simulink model "spherical_wrist"  (R2023b)
settings: Solver=VariableStepAuto  StartTime=0.0  StopTime=20  FixedStep=0.001  RelTol=1e-3
InitFcn:
  | WRIST_60_50_DataFile
model workspace (MAT data in the model file):
  Damp = Simulink.Parameter
  Damp.Value = 0.0001
  Damp.DataType = 'auto'
  Damp.Complexity = 'real'
  Damp.Dimensions = [1 1]
  Dm = Simulink.Parameter
  Dm.Value = 7.4e-05
  Dm.DataType = 'auto'
  Dm.DocUnits = 'mN*m/rpm'
  Dm.Complexity = 'real'
  Dm.Dimensions = [1 1]
  Jm = Simulink.Parameter
  Jm.Value = 3.3
  Jm.DataType = 'auto'
  Jm.DocUnits = 'g*cm^2'
  Jm.Complexity = 'real'
  Jm.Dimensions = [1 1]
  Km = Simulink.Parameter
  Km.Value = 32.2
  Km.DataType = 'auto'
  Km.DocUnits = 'mN*m/A'
  Km.Complexity = 'real'
  Km.Dimensions = [1 1]
  Tc = Simulink.Parameter
  Tc.Value = 0.001
  Tc.DataType = 'auto'
  Tc.DocUnits = 's'
  Tc.Complexity = 'real'
  Tc.Dimensions = [1 1]
values from neighbouring files (symbols this model uses):
  PQ = [P(1,:)*Q(1,:)' P(2,:)*Q(2,:)' P(3,:)*Q(3,:)']    [WRIST_60_50_DataFile.m]
  Pz = -tand(30)*[1; 1; 1]    [WRIST_60_50_DataFile.m]
  Q = [cosd(plat_off) sind(plat_off) [0; 0; 0]]    [WRIST_60_50_DataFile.m]
undefined symbols (not defined in the file or in its folder): smiData, X, Y, Z
libraries: sm_lib x44, nesl_utility x20, fl_lib x15, sdl_lib x9, sharedtransform x2, slpidlib x1
(part 1 of 3)
settings Model: Creator=ascalzo  LastModifiedBy=upattacini
settings SolverCC: AlgebraicLoopSolver=TrustRegion
settings OptimizationCC: DefaultParameterBehavior=Inlined  UseDivisionForNetSlopeComputation=on  GainParamInheritBuiltInType=on  UseFloatMulNetSlope=on  InlineInvariantSignals=on  ReuseModelBlockBuffer=off  PassReuseOutputArgsAs=Individual arguments  ZeroExternalMemoryAtStartup=off  ZeroInternalMemoryAtStartup=off  NoFixptDivByZeroProtection=on  EfficientFloat2IntCast=on  LifeSpan=1  OptimizeBlockOrder=speed  DifferentSizesBufferReuse=on  EfficientTunableParamExpr=on
settings DebuggingCC: ParameterTunabilityLossMsg=error  UnconnectedInputMsg=warning  UnconnectedOutputMsg=warning  UnconnectedLineMsg=warning
settings HardwareCC: ProdBitPerPointer=32  ProdBitPerSizeT=32  ProdBitPerPtrDiffT=32  ProdLargestAtomicInteger=Long  ProdLargestAtomicFloat=Double  ProdWordSize=32  ProdLongLongMode=on  ProdHWDeviceType=ARM Compatible->ARM Cortex-M
settings ModelReferenceCC: EnableRefExpFcnMdlSchedulingChecks=on
settings SFSimCC: MATLABDynamicMemAlloc=off  SimTargetLang=C++
settings RTWCC: Description=Embedded Coder  SystemTargetFile=ert.tlc  GenCodeOnly=on  PackageGeneratedCodeAndArtifacts=on  PackageName=WristDecoupler.zip  TemplateMakefile=ert_default_tmf  GenerateReport=on  Toolchain=Microsoft Visual C++ 2019 v16.0 | nmake (64-bit Windows)  LaunchReport=on  TargetLang=C++  DLArmComputeVersion=19.05
settings CodeAppCC: ForceParamTrailComments=on  IgnoreCustomStorageClasses=off  OperatorAnnotations=on  SimulinkDataObjDesc=on  SFDataObjDesc=on  CustomSymbolStrGlobalVar=rt$N$M  CustomSymbolStrType=$N$M  CustomSymbolStrFcn=$N$M$F  CustomSymbolStrMacro=$N$M  InsertBlockDesc=on  MATLABSourceComments=on
settings ERTTargetCC: TargetLangStandard=C++03 (ISO)  GenerateSampleERTMain=on  IncludeMdlTerminateFcn=off  CombineSignalStateStructs=on  CodeInterfacePackaging=C++ class  SupportComplex=off  SupportNonInlinedSFcns=on  InlinedParameterPlacement=NonHierarchical  RootIOFormat=Structure reference  ERTCustomFileTemplate=example_file_process.tlc  ERTFilePackagingFormat=CompactWithDataFile

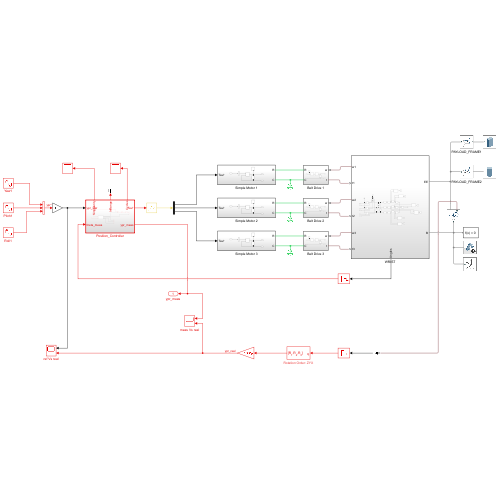
[thumbnail: Simulink's stored preview of the top-level diagram]
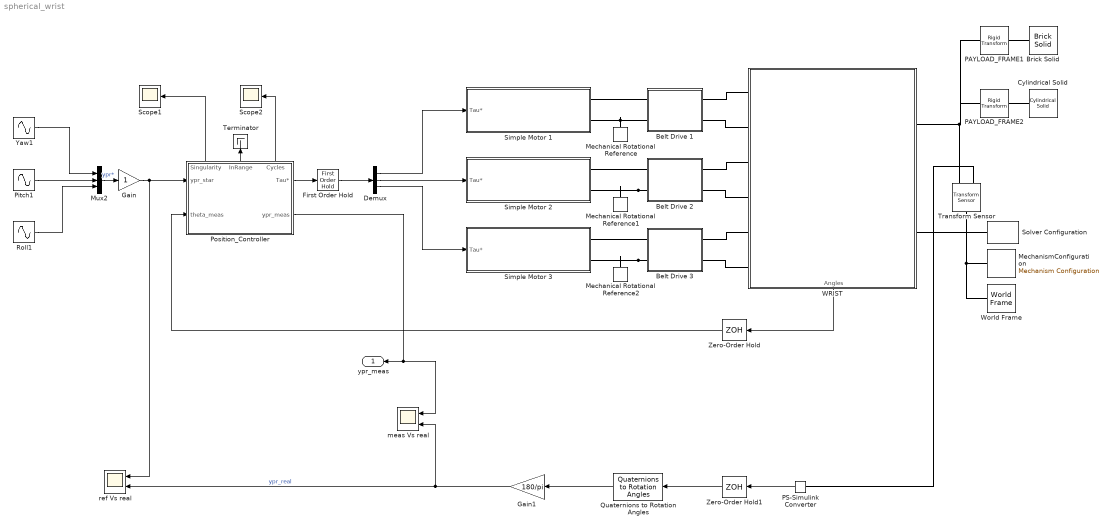
== system spherical_wrist ==
  Belt Drive 1 : Subsystem
  Belt Drive 2 : Subsystem
  Belt Drive 3 : Subsystem
  Brick Solid : sm_lib/Body Elements/Brick Solid  GraphicAmbientColor=[0.15 0.15 0.15 1.0]  BasedOnType=Density  BrickDimensions=[50 50 50]  BrickDimensionsUnits=mm  CenterOfMass=[0 0 0]  CenterOfMassUnits=m  GraphicDiffuseColor=[0.5 0.5 0.5]  Density=12000  DensityUnits=kg/m^3  DoExposeReferenceFrame=on  GraphicEmissiveColor=[0.0 0.0 0.0 1.0]  ExportEntireGeometry=off  SerializedFrames=<Frames/>  MarkerShape=Sphere  MarkerSize=10  GraphicType=FromGeometry  InertiaType=CalculateFromGeometry  Mass=1.5  MassUnits=kg  MomentsOfInertia=[1 1 1]  MomentsOfInertiaUnits=kg*m^2  GraphicOpacity=1  ProductsOfInertia=[0 0 0]  ProductsOfInertiaUnits=kg*m^2  GraphicShininess=75  GraphicSpecularColor=[0.5 0.5 0.5 1.0]  GraphicVisPropType=SimpleVisualProperties
  Cylindrical Solid : sm_lib/Body Elements/Cylindrical Solid  GraphicAmbientColor=[0.15 0.15 0.15 1.0]  BasedOnType=Density  CenterOfMass=[0 0 0]  CenterOfMassUnits=m  GraphicDiffuseColor=[0.5 0.5 0.5]  CylinderLength=56  CylinderLengthUnits=mm  CylinderRadius=4  CylinderRadiusUnits=mm  Density=1000  DensityUnits=kg/m^3  DoExposeReferenceFrame=on  GraphicEmissiveColor=[0.0 0.0 0.0 1.0]  ExportEntireGeometry=off  SerializedFrames=<Frames/>  MarkerShape=Sphere  MarkerSize=10  GraphicType=FromGeometry  InertiaType=PointMass  Mass=500  MassUnits=g  MomentsOfInertia=[1 1 1]  MomentsOfInertiaUnits=kg*m^2  GraphicOpacity=1  ProductsOfInertia=[0 0 0]  ProductsOfInertiaUnits=kg*m^2  GraphicShininess=75  GraphicSpecularColor=[0.5 0.5 0.5 1.0]  GraphicVisPropType=SimpleVisualProperties
  Demux : Demux  Outputs=3
  First Order Hold : FirstOrderHold  ErrorTolerance=inf
  Gain : Gain
  Gain1 : Gain  Gain=180/pi
  Mechanical Rotational Reference : fl_lib/Mechanical/Rotational Elements/Mechanical Rotational Reference
  Mechanical Rotational Reference1 : fl_lib/Mechanical/Rotational Elements/Mechanical Rotational Reference
  Mechanical Rotational Reference2 : fl_lib/Mechanical/Rotational Elements/Mechanical Rotational Reference
  MechanismConfiguration : sm_lib/Utilities/Mechanism Configuration  UniformGravity=Constant  GravityVector=[0 0 9.80665]  GravityVectorUnits=m/s^2  LinearizationDelta=0.001  JointModeTransitionNonlinearIterations=2
  Mux2 : Mux  Inputs=3
  PAYLOAD_FRAME1 : sm_lib/Frames and Transforms/Rigid Transform  TranslationMethod=Cartesian  TranslationStandardOffset=0  TranslationStandardOffsetUnits=mm  TranslationStandardAxis=+Z  TranslationCartesianOffset=[0 0 70]  TranslationCartesianOffsetUnits=mm  TranslationROffset=0  TranslationROffsetUnits=m  TranslationZOffset=0  TranslationZOffsetUnits=m  TranslationThetaOffset=0  TranslationThetaOffsetUnits=deg  RotationMethod=None  RotationAngleUnits=rad  RotationStandardAxis=+Z  RotationAngle=smiData.RigidTransform(2).angle  RotationArbitraryAxis=smiData.RigidTransform(2).axis  FollAlignAxisA=+X  BaseAlignAxisA=+Y  FollAlignAxisB=+Y  BaseAlignAxisB=+Z  RotationSequenceAxes=FollowerAxes  RotationSequence=XYX  RotationSequenceAngles=[0 0 0]  RotationSequenceAnglesUnits=deg  RotationMatrix=[1 0 0; 0 1 0; 0 0 1]  Quaternion=[1 0 0 0]
  PAYLOAD_FRAME2 : sm_lib/Frames and Transforms/Rigid Transform  TranslationMethod=Cartesian  TranslationStandardOffset=0  TranslationStandardOffsetUnits=mm  TranslationStandardAxis=+Z  TranslationCartesianOffset=[0 0 30]  TranslationCartesianOffsetUnits=mm  TranslationROffset=0  TranslationROffsetUnits=m  TranslationZOffset=0  TranslationZOffsetUnits=m  TranslationThetaOffset=0  TranslationThetaOffsetUnits=deg  RotationMethod=None  RotationAngleUnits=rad  RotationStandardAxis=+Z  RotationAngle=smiData.RigidTransform(2).angle  RotationArbitraryAxis=smiData.RigidTransform(2).axis  FollAlignAxisA=+X  BaseAlignAxisA=+Y  FollAlignAxisB=+Y  BaseAlignAxisB=+Z  RotationSequenceAxes=FollowerAxes  RotationSequence=XYX  RotationSequenceAngles=[0 0 0]  RotationSequenceAnglesUnits=deg  RotationMatrix=[1 0 0; 0 1 0; 0 0 1]  Quaternion=[1 0 0 0]
  PS-Simulink Converter : nesl_utility/PS-Simulink Converter  PhysicalDomain=network_engine_domain  SubClassName=ps_output  LeftPortType=input  RightPortType=output  PseudoPeriodic=off  Frequencies=[]  VectorFormat=1-D array  Unit=inherit  AffineConversion=off
  Pitch1 : Sin  Amplitude=55  Bias=-5  Frequency=60/55  Phase=asin(5/55)  SampleTime=Tc
  Position_Controller : Subsystem  TreatAsAtomicUnit=on  SystemSampleTime=0.001
      settings: MinAlgLoopOccurrences=on  PortSchema="{\"entries\":[{\"content\":{\"sides\":[{\"content\":{\"connectorIds\":[\"In1\",\"In2\"]},\"type\":\"ConnectorPlacement.EquallySpacedRectSide\",\"uuid\":\"83213a6a-d539-4d4b-893d-998d212c9f51\"},{\"content\":{\"connectorIds\":[\"Out1\",\"Out2\"],\"side\":\"RIGHT\"},\"type\":\"ConnectorPlacement.EquallySpacedRectSide\",\"uuid\":\"07d19463-f1b8-4ef2-82ae-a356a5259b0c\"},{\"content\":{\"connectorIds\":[\"Out3\",\"Out4\",\"Out5\"],\"side\":\"TOP\"},\"type\":\"ConnectorPlacement.EquallySpacedRectSide\",\"uuid\":\"262960f5-5579-40eb-9028-5284e67b897c\"}]},\"type\":\"ConnectorPlacement.EquallySpacedConnector\",\"uuid\":\"3a54d725-4b36-4299-8af9-8f83752d9c8a\"}],\"packageUris\":[\"http://schema.mathworks.com/mf0/Connector/19700101\"],\"version\":\"1.0\"}"
  Quaternions to Rotation Angles : sharedtransform/Quaternions to Rotation Angles  rotationOrder=ZYX  aMode=aMode
  Roll1 : Sin  Amplitude=30  Frequency=60/30  SampleTime=Tc
  Scope1 : Scope
  Scope2 : Scope
  Simple Motor 1 : Subsystem
  Simple Motor 2 : Subsystem
  Simple Motor 3 : Subsystem
  Solver Configuration : nesl_utility/Solver Configuration  PhysicalDomain=network_engine_domain  SubClassName=solver  LeftPortType=input  RightPortType=generic  Tones=[]  Harmonics=[]  SimulateNoise=off  Profile=off  UseLocalSampling=off  EnableSwitchedLinearOptims=on  FrequencyDomain=off  UseCCode=off  RelTol=0.001  AbsTol=1e-06  MinStep=1e-09  ToWorkspace=off  RevertToSquareIcSolve=off  NumHomotopyIterations=100  PhasorMode=off  PhasorModeNumHarmonics=1  ConsistencySolver=NEWTON_FTOL  IndexReductionMethod=DerivativeReplacement  DoDC=off  ResidualTolerance=1e-09  ConsistencyTolSource=GLOBAL  ConsistencyAbsTol=0.001  ConsistencyRelTol=0.001  ConsistencyTolFactor=0.001  UseLocalSolver=off  LocalSolverChoice=NE_TRAPEZOIDAL_ADVANCER  ResolveIndetEquations=on  FunctionEvalNumThread=1  LocalSolverSampleTime=0.0001  DoFixedCost=off  MaxNonlinIter=3  MaxModeIter=2  ComputeImpulses=off  ImpulseIterations=2  LinearAlgebra=auto  LinearAlgebraNumThread=0  EquationFormulation=NE_TIME_EF  DelaysMemoryBudget=1024  AutomaticFiltering=on  FilteringTimeConstant=0.001  PartitionStorageMethod=AS_NEEDED  PartitionMemoryBudget=1024  PartitionMethod=ROBUST  MultibodyUseLocalSolver=off  MultibodyLocalSolverChoice=ODE1  MultibodyLocalSolverSampleTime=0.001
  Terminator : Terminator
  Transform Sensor : sm_lib/Frames and Transforms/Transform Sensor  MeasurementFrame=World  RotationSequence=XYX  SenseAngle=off  SenseAxis=off  SenseQ=on  SenseR=off  SenseRotationSequence=off  SenseOmegaX=off  SenseOmegaY=off  SenseOmegaZ=off  SenseOmega=off  SenseQDot=off  SenseRDot=off  SenseRotationSequenceDot=off  SenseAlphaX=off  SenseAlphaY=off  SenseAlphaZ=off  SenseAlpha=off  SenseQDDot=off  SenseRDDot=off  SenseX=off  SenseY=off  SenseZ=off  SenseXYZ=off  SenseRad=off  SenseAzim=off  SenseDist=off  SenseInc=off  SenseXDot=off  SenseYDot=off  SenseZDot=off  SenseXYZDot=off  SenseRadDot=off  SenseAzimDot=off  SenseDistDot=off  SenseIncDot=off  SenseXDDot=off  SenseYDDot=off  SenseZDDot=off  SenseXYZDDot=off  SenseRadDDot=off  SenseAzimDDot=off  SenseDistDDot=off  SenseIncDDot=off
  WRIST : Subsystem
      settings: PortSchema="{\"entries\":[{\"content\":{\"sides\":[{\"content\":{\"connectorIds\":[\"LConn1\",\"LConn2\",\"LConn3\",\"LConn4\",\"LConn5\",\"LConn6\"]},\"type\":\"ConnectorPlacement.EquallySpacedRectSide\",\"uuid\":\"837cba77-e4d8-410a-871c-09f9d5b58985\"},{\"content\":{\"connectorIds\":[\"RConn1\",\"RConn2\"],\"side\":\"RIGHT\"},\"type\":\"ConnectorPlacement.EquallySpacedRectSide\",\"uuid\":\"e99e27fa-5cde-4df4-999c-5c540dbd874f\"},{\"content\":{\"connectorIds\":[],\"side\":\"TOP\"},\"type\":\"ConnectorPlacement.EquallySpacedRectSide\",\"uuid\":\"93dbe70b-6d44-4b10-9b14-70f8e934205d\"},{\"content\":{\"connectorIds\":[\"Out1\"],\"side\":\"BOTTOM\"},\"type\":\"ConnectorPlacement.EquallySpacedRectSide\",\"uuid\":\"bafba6b5-af66-4d82-b4b8-19931a0ab184\"}]},\"type\":\"ConnectorPlacement.EquallySpacedConnector\",\"uuid\":\"c57b24f6-44a7-49b3-8fbc-a4c709c10c31\"}],\"packageUris\":[\"http://schema.mathworks.com/mf0/Connector/19700101\"],\"version\":\"1.0\"}"
  World Frame : sm_lib/Frames and Transforms/World Frame
  Yaw1 : Sin  Amplitude=90  Frequency=60/90  SampleTime=Tc
  Zero-Order Hold : ZeroOrderHold  SampleTime=Tc
  Zero-Order Hold1 : ZeroOrderHold  SampleTime=Tc
  meas Vs real : Scope  NumInputPorts=2
  ref Vs real : Scope  NumInputPorts=2
  ypr_meas : Outport
  wires:
  WRIST/1(Angles) -> Zero-Order Hold/1
  Gain1/1 -> ref Vs real/2, meas Vs real/2  "ypr_real"
  PS-Simulink Converter/1 -> Zero-Order Hold1/1
  Quaternions to Rotation Angles/1 -> Gain1/1
  Yaw1/1 -> Mux2/1
  Mux2/1 -> Gain/1  "ypr*"
  Roll1/1 -> Mux2/3
  Pitch1/1 -> Mux2/2
  Demux/1 -> Simple Motor 1/1(Tau*)
  Demux/2 -> Simple Motor 2/1(Tau*)
  Demux/3 -> Simple Motor 3/1(Tau*)
  First Order Hold/1 -> Demux/1
  Position_Controller/2(ypr_meas) -> meas Vs real/1, ypr_meas/1
  Position_Controller/1(Tau*) -> First Order Hold/1
  Position_Controller/5(Cycles) -> Scope2/1
  Gain/1 -> ref Vs real/1, Position_Controller/1(ypr_star)
  Position_Controller/3(Singularity) -> Scope1/1
  Position_Controller/4(InRange) -> Terminator/1
  Zero-Order Hold/1 -> Position_Controller/2(theta_meas)
  Zero-Order Hold1/1 -> Quaternions to Rotation Angles/1
  connections:
  World Frame/RConn1 -- Solver Configuration/RConn1 -- Transform Sensor/LConn1 -- WRIST/RConn2 -- MechanismConfiguration/RConn1
  PAYLOAD_FRAME1/LConn1 -- PAYLOAD_FRAME2/LConn1 -- Transform Sensor/RConn1 -- WRIST/RConn1
  Transform Sensor/RConn2 -- PS-Simulink Converter/LConn1
  Cylindrical Solid/RConn1 -- PAYLOAD_FRAME2/RConn1
  Brick Solid/RConn1 -- PAYLOAD_FRAME1/RConn1
  WRIST/LConn1 -- Belt Drive 1/RConn1
  Mechanical Rotational Reference/LConn1 -- Simple Motor 1/RConn2 -- Belt Drive 1/LConn2
  Belt Drive 1/LConn1 -- Simple Motor 1/RConn1
  Belt Drive 2/LConn2 -- Simple Motor 2/RConn2 -- Mechanical Rotational Reference1/LConn1
  Belt Drive 2/LConn1 -- Simple Motor 2/RConn1
  WRIST/LConn3 -- Belt Drive 2/RConn1
  Belt Drive 3/LConn2 -- Simple Motor 3/RConn2 -- Mechanical Rotational Reference2/LConn1
  Belt Drive 3/LConn1 -- Simple Motor 3/RConn1
  WRIST/LConn5 -- Belt Drive 3/RConn1
  Belt Drive 1/RConn2 -- WRIST/LConn2
  Belt Drive 2/RConn2 -- WRIST/LConn4
  Belt Drive 3/RConn2 -- WRIST/LConn6

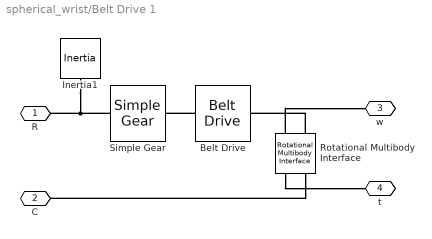
== system spherical_wrist/Belt Drive 1 ==
  Belt Drive : sdl_lib/Couplings & Drives/Belt Drive  drive_type=sdl.enum.wrap_configuration.open  belt_type=sdl.enum.belt_type.ideal  sheave_ang=30 deg  num_belts=1  model_f_c=sdl.enum.model_centrifugal.off  linear_density=0.6 kg/m  model_compliance=sdl.enum.compliance.off  stiffness=1e4 N/m  damping=1e3 N/(m/s)  tension=100 N  breakable=sdl.enum.max_tension.off  F_max=1e5 N  r_pulley_A=14 mm  b_pulley_A=0.1 N*m/(rad/s)  model_inertia_A=sdl.enum.model_inertia.on  pulley_inertia_A=10 g*mm^2  initial_velocity_A=0 rad/s  r_pulley_B=28 mm  b_pulley_B=0.1 N*m/(rad/s)  model_inertia_B=sdl.enum.model_inertia.on  pulley_inertia_B=10 g*mm^2  initial_velocity_B=0 rad/s  friction_model=sdl.enum.PulleyModel.Continuous  initial_state_locked_A=sdl.enum.initial_lock.unlocked  initial_state_locked_B=sdl.enum.initial_lock.unlocked  mu=0.5  mu_static=0.5  mu_kinetic=0.42  wrap_parameterization=sdl.enum.wrap_parameterization.centers  d_centers=0.5 m  phi_wrap_A=145 deg  phi_wrap_B=215 deg  v_thr=0.001 m/s  f_thr=1 N
      settings: InternalSimscapePortConfiguration="{\"Bottom\":[],\"Left\":[{\"id\":\"A\",\"label\":\"A\",\"type\":\"foundation.mechanical.rotational.rotational\"}],\"Right\":[{\"id\":\"B\",\"label\":\"B\",\"type\":\"foundation.mechanical.rotational.rotational\"}],\"Top\":[]}"
  Inertia1 : fl_lib/Mechanical/Rotational Elements/Inertia  inertia=34 g*mm^2  num_ports=foundation.enum.numPorts2.one  w_specify=off  w_priority=High  w=0 rad/s  w_nominal_specify=off  w_nominal_unit=rad/s  w_nominal_value=1  t_specify=off  t_priority=None  t=0 N*m  t_nominal_specify=off  t_nominal_unit=N*m  t_nominal_value=1
  Rotational Multibody Interface : fl_lib/Mechanical/Multibody Interfaces/Rotational Multibody Interface
  Simple Gear : sdl_lib/Gears/Simple Gear  ratio=196  rotation_direction=3-2*(1)  friction_model=sdl.enum.gear_efficiencies_load.constant  T_noload=0.1 N*m  T_nom=5 N*m  efficiency_nom=0.8  efficiency=0.78  temperature_TLU=[280, 300, 320] K  load_TLU=[1, 5, 10] N*m  efficiency_TLU=[.95, .9, .85]  efficiency_TLU2=[.85, .8, .75; .95, .9, .85; .85, .8, .7]  w_thr=0.01 rad/s  pwr_thr=9 W  enable_backlash=false  hardstop_model=simscape.enum.hardstop.smooth  backlash_distance=1e-3 mm  r_base=0.1 m  transition=1e-4 mm  backlash_stiffness=1e7 N/m  backlash_damping=1e6 N*s/m  coeff_rest=0  v_tol=0.001 m/s  f_tol=0 N  mu_visc=[0, 0] N*m/(rad/s)  enable_faults=simscape.enum.onoff.off  efficiency_fault=0.05  external_fault=simscape.enum.onoff.off  temporal_fault=simscape.enum.onoff.off  fault_time=5 s  fault_angles=pi / 12 rad  report_fault=(1)-1  thermal_mass=50 J/K  temperature_specify=off  temperature_priority=High  temperature=300 K  temperature_nominal_specify=off  temperature_nominal_unit=K  temperature_nominal_value=1  x_backlash_specify=off  x_backlash_priority=None  x_backlash=0 mm  x_backlash_nominal_specify=off  x_backlash_nominal_unit=mm  x_backlash_nominal_value=1  f_hardstop_specify=off  f_hardstop_priority=None  f_hardstop=0 N  f_hardstop_nominal_specify=off  f_hardstop_nominal_unit=N  f_hardstop_nominal_value=1  v_backlash_specify=off  v_backlash_priority=None  v_backlash=0 m/s  v_backlash_nominal_specify=off  v_backlash_nominal_unit=m/s  v_backlash_nominal_value=1
  R : PMIOPort  Side=Left
  C : PMIOPort  Port=2  Side=Left
  w : PMIOPort  Port=3  Side=Right
  t : PMIOPort  Port=4  Side=Right
  connections:
  Rotational Multibody Interface/RConn2 -- Belt Drive/RConn1
  Simple Gear/LConn1 -- R/RConn1 -- Inertia1/LConn1
  Rotational Multibody Interface/RConn1 -- w/RConn1
  Belt Drive/LConn1 -- Simple Gear/RConn1
  Rotational Multibody Interface/LConn1 -- t/RConn1
  Rotational Multibody Interface/LConn2 -- C/RConn1

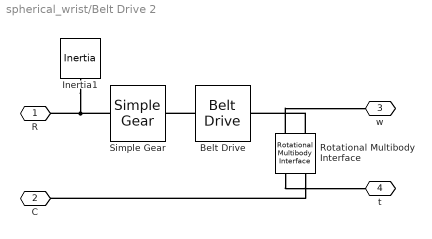
== system spherical_wrist/Belt Drive 2 ==
  Belt Drive : sdl_lib/Couplings & Drives/Belt Drive  drive_type=sdl.enum.wrap_configuration.open  belt_type=sdl.enum.belt_type.ideal  sheave_ang=30 deg  num_belts=1  model_f_c=sdl.enum.model_centrifugal.off  linear_density=0.6 kg/m  model_compliance=sdl.enum.compliance.off  stiffness=1e4 N/m  damping=1e3 N/(m/s)  tension=100 N  breakable=sdl.enum.max_tension.off  F_max=1e5 N  r_pulley_A=14 mm  b_pulley_A=0.1 N*m/(rad/s)  model_inertia_A=sdl.enum.model_inertia.on  pulley_inertia_A=10 g*mm^2  initial_velocity_A=0 rad/s  r_pulley_B=28 mm  b_pulley_B=0.1 N*m/(rad/s)  model_inertia_B=sdl.enum.model_inertia.on  pulley_inertia_B=10 g*mm^2  initial_velocity_B=0 rad/s  friction_model=sdl.enum.PulleyModel.Continuous  initial_state_locked_A=sdl.enum.initial_lock.unlocked  initial_state_locked_B=sdl.enum.initial_lock.unlocked  mu=0.5  mu_static=0.5  mu_kinetic=0.42  wrap_parameterization=sdl.enum.wrap_parameterization.centers  d_centers=0.5 m  phi_wrap_A=145 deg  phi_wrap_B=215 deg  v_thr=0.001 m/s  f_thr=1 N
      settings: InternalSimscapePortConfiguration="{\"Bottom\":[],\"Left\":[{\"id\":\"A\",\"label\":\"A\",\"type\":\"foundation.mechanical.rotational.rotational\"}],\"Right\":[{\"id\":\"B\",\"label\":\"B\",\"type\":\"foundation.mechanical.rotational.rotational\"}],\"Top\":[]}"
  Inertia1 : fl_lib/Mechanical/Rotational Elements/Inertia  inertia=34 g*mm^2  num_ports=foundation.enum.numPorts2.one  w_specify=off  w_priority=High  w=0 rad/s  w_nominal_specify=off  w_nominal_unit=rad/s  w_nominal_value=1  t_specify=off  t_priority=None  t=0 N*m  t_nominal_specify=off  t_nominal_unit=N*m  t_nominal_value=1
  Rotational Multibody Interface : fl_lib/Mechanical/Multibody Interfaces/Rotational Multibody Interface
  Simple Gear : sdl_lib/Gears/Simple Gear  ratio=196  rotation_direction=3-2*(1)  friction_model=sdl.enum.gear_efficiencies_load.constant  T_noload=0.1 N*m  T_nom=5 N*m  efficiency_nom=0.8  efficiency=0.78  temperature_TLU=[280, 300, 320] K  load_TLU=[1, 5, 10] N*m  efficiency_TLU=[.95, .9, .85]  efficiency_TLU2=[.85, .8, .75; .95, .9, .85; .85, .8, .7]  w_thr=0.01 rad/s  pwr_thr=9 W  enable_backlash=false  hardstop_model=simscape.enum.hardstop.smooth  backlash_distance=1e-3 mm  r_base=0.1 m  transition=1e-4 mm  backlash_stiffness=1e7 N/m  backlash_damping=1e6 N*s/m  coeff_rest=0  v_tol=0.001 m/s  f_tol=0 N  mu_visc=[0, 0] N*m/(rad/s)  enable_faults=simscape.enum.onoff.off  efficiency_fault=0.05  external_fault=simscape.enum.onoff.off  temporal_fault=simscape.enum.onoff.off  fault_time=5 s  fault_angles=pi / 12 rad  report_fault=(1)-1  thermal_mass=50 J/K  temperature_specify=off  temperature_priority=High  temperature=300 K  temperature_nominal_specify=off  temperature_nominal_unit=K  temperature_nominal_value=1  x_backlash_specify=off  x_backlash_priority=None  x_backlash=0 mm  x_backlash_nominal_specify=off  x_backlash_nominal_unit=mm  x_backlash_nominal_value=1  f_hardstop_specify=off  f_hardstop_priority=None  f_hardstop=0 N  f_hardstop_nominal_specify=off  f_hardstop_nominal_unit=N  f_hardstop_nominal_value=1  v_backlash_specify=off  v_backlash_priority=None  v_backlash=0 m/s  v_backlash_nominal_specify=off  v_backlash_nominal_unit=m/s  v_backlash_nominal_value=1
  R : PMIOPort  Side=Left
  C : PMIOPort  Port=2  Side=Left
  w : PMIOPort  Port=3  Side=Right
  t : PMIOPort  Port=4  Side=Right
  connections:
  Rotational Multibody Interface/RConn2 -- Belt Drive/RConn1
  Inertia1/LConn1 -- Simple Gear/LConn1 -- R/RConn1
  Rotational Multibody Interface/RConn1 -- w/RConn1
  Belt Drive/LConn1 -- Simple Gear/RConn1
  Rotational Multibody Interface/LConn1 -- t/RConn1
  Rotational Multibody Interface/LConn2 -- C/RConn1

== system spherical_wrist/Belt Drive 3 ==
  Belt Drive : sdl_lib/Couplings & Drives/Belt Drive  drive_type=sdl.enum.wrap_configuration.open  belt_type=sdl.enum.belt_type.ideal  sheave_ang=30 deg  num_belts=1  model_f_c=sdl.enum.model_centrifugal.off  linear_density=0.6 kg/m  model_compliance=sdl.enum.compliance.off  stiffness=1e4 N/m  damping=1e3 N/(m/s)  tension=100 N  breakable=sdl.enum.max_tension.off  F_max=1e5 N  r_pulley_A=14 mm  b_pulley_A=0.1 N*m/(rad/s)  model_inertia_A=sdl.enum.model_inertia.on  pulley_inertia_A=10 g*mm^2  initial_velocity_A=0 rad/s  r_pulley_B=28 mm  b_pulley_B=0.1 N*m/(rad/s)  model_inertia_B=sdl.enum.model_inertia.on  pulley_inertia_B=10 g*mm^2  initial_velocity_B=0 rad/s  friction_model=sdl.enum.PulleyModel.Continuous  initial_state_locked_A=sdl.enum.initial_lock.unlocked  initial_state_locked_B=sdl.enum.initial_lock.unlocked  mu=0.5  mu_static=0.5  mu_kinetic=0.42  wrap_parameterization=sdl.enum.wrap_parameterization.centers  d_centers=0.5 m  phi_wrap_A=145 deg  phi_wrap_B=215 deg  v_thr=0.001 m/s  f_thr=1 N
      settings: InternalSimscapePortConfiguration="{\"Bottom\":[],\"Left\":[{\"id\":\"A\",\"label\":\"A\",\"type\":\"foundation.mechanical.rotational.rotational\"}],\"Right\":[{\"id\":\"B\",\"label\":\"B\",\"type\":\"foundation.mechanical.rotational.rotational\"}],\"Top\":[]}"
  Inertia1 : fl_lib/Mechanical/Rotational Elements/Inertia  inertia=34 g*mm^2  num_ports=foundation.enum.numPorts2.one  w_specify=off  w_priority=High  w=0 rad/s  w_nominal_specify=off  w_nominal_unit=rad/s  w_nominal_value=1  t_specify=off  t_priority=None  t=0 N*m  t_nominal_specify=off  t_nominal_unit=N*m  t_nominal_value=1
  Rotational Multibody Interface : fl_lib/Mechanical/Multibody Interfaces/Rotational Multibody Interface
  Simple Gear : sdl_lib/Gears/Simple Gear  ratio=196  rotation_direction=3-2*(1)  friction_model=sdl.enum.gear_efficiencies_load.constant  T_noload=0.1 N*m  T_nom=5 N*m  efficiency_nom=0.8  efficiency=0.78  temperature_TLU=[280, 300, 320] K  load_TLU=[1, 5, 10] N*m  efficiency_TLU=[.95, .9, .85]  efficiency_TLU2=[.85, .8, .75; .95, .9, .85; .85, .8, .7]  w_thr=0.01 rad/s  pwr_thr=9 W  enable_backlash=false  hardstop_model=simscape.enum.hardstop.smooth  backlash_distance=1e-3 mm  r_base=0.1 m  transition=1e-4 mm  backlash_stiffness=1e7 N/m  backlash_damping=1e6 N*s/m  coeff_rest=0  v_tol=0.001 m/s  f_tol=0 N  mu_visc=[0, 0] N*m/(rad/s)  enable_faults=simscape.enum.onoff.off  efficiency_fault=0.05  external_fault=simscape.enum.onoff.off  temporal_fault=simscape.enum.onoff.off  fault_time=5 s  fault_angles=pi / 12 rad  report_fault=(1)-1  thermal_mass=50 J/K  temperature_specify=off  temperature_priority=High  temperature=300 K  temperature_nominal_specify=off  temperature_nominal_unit=K  temperature_nominal_value=1  x_backlash_specify=off  x_backlash_priority=None  x_backlash=0 mm  x_backlash_nominal_specify=off  x_backlash_nominal_unit=mm  x_backlash_nominal_value=1  f_hardstop_specify=off  f_hardstop_priority=None  f_hardstop=0 N  f_hardstop_nominal_specify=off  f_hardstop_nominal_unit=N  f_hardstop_nominal_value=1  v_backlash_specify=off  v_backlash_priority=None  v_backlash=0 m/s  v_backlash_nominal_specify=off  v_backlash_nominal_unit=m/s  v_backlash_nominal_value=1
  R : PMIOPort  Side=Left
  C : PMIOPort  Port=2  Side=Left
  w : PMIOPort  Port=3  Side=Right
  t : PMIOPort  Port=4  Side=Right
  connections:
  Rotational Multibody Interface/RConn2 -- Belt Drive/RConn1
  Inertia1/LConn1 -- Simple Gear/LConn1 -- R/RConn1
  Rotational Multibody Interface/RConn1 -- w/RConn1
  Belt Drive/LConn1 -- Simple Gear/RConn1
  Rotational Multibody Interface/LConn1 -- t/RConn1
  Rotational Multibody Interface/LConn2 -- C/RConn1

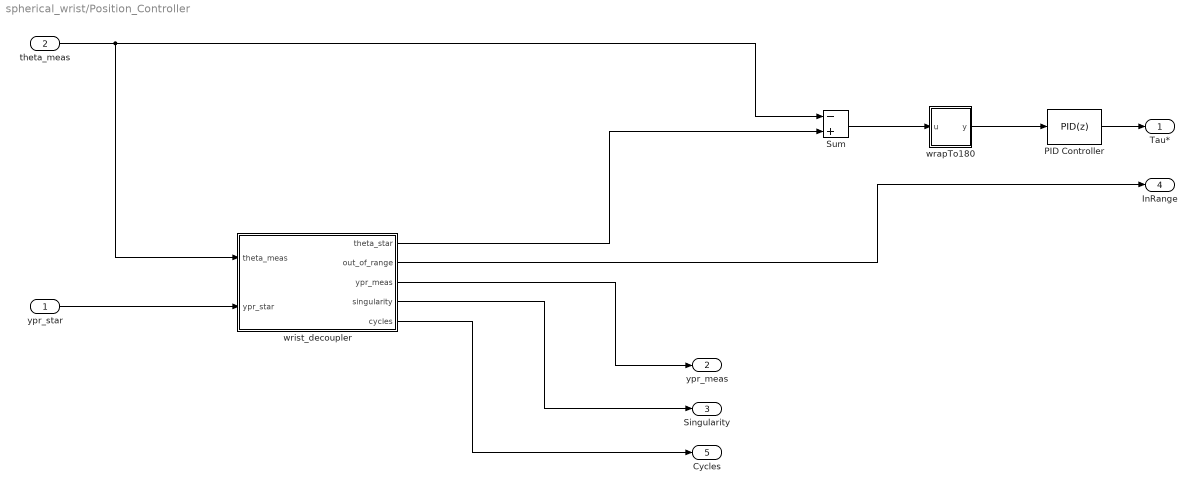
== system spherical_wrist/Position_Controller ==
  ypr_star : Inport
  theta_meas : Inport  Port=2
  PID Controller : slpidlib/PID Controller  Controller=PID  Form=Ideal  TimeDomain=Discrete-time  UseExternalTs=off  SampleTime=-1  IntegratorMethod=Forward Euler  FilterMethod=Forward Euler  ControllerParametersSource=internal  P=1/200  I=0.5  UseKiTs=off  D=0.0125  N=100  UseFilter=on  TunerSelectOption=Transfer Function Based (PID Tuner App)  InitialConditionSource=internal  InitialConditionForIntegrator=0  InitialConditionForFilter=0  DifferentiatorICPrevScaledInput=0  ExternalReset=none  TrackingMode=off  Kt=1  LimitOutput=on  SatLimitsSource=internal  UpperSaturationLimit=0.0102*3  LowerSaturationLimit=-0.0102*3  LinearizeAsGain=on  AntiWindupMode=clamping  Kb=1  LimitIntegrator=off  UpperIntegratorSaturationLimit=inf  LowerIntegratorSaturationLimit=-inf  POutMin=[]  POutMax=[]  IOutMin=[]  IOutMax=[]  DOutMin=[]  DOutMax=[]  NOutMin=[]  NOutMax=[]  SumOutMin=[]  SumOutMax=[]  SaturationOutMin=[]  SaturationOutMax=[]  PParamMin=[]  PParamMax=[]  IParamMin=[]  IParamMax=[]  DParamMin=[]  DParamMax=[]  NParamMin=[]  NParamMax=[]  KbParamMin=[]  KbParamMax=[]  KtParamMin=[]  KtParamMax=[]  KbOutMin=[]  KbOutMax=[]  KtOutMin=[]  KtOutMax=[]  IntegratorOutMin=[]  IntegratorOutMax=[]  FilterOutMin=[]  FilterOutMax=[]  SumI1OutMin=[]  SumI1OutMax=[]  SumI2OutMin=[]  SumI2OutMax=[]  SumI3OutMin=[]  SumI3OutMax=[]  SumI4OutMin=[]  SumI4OutMax=[]  SumDOutMin=[]  SumDOutMax=[]  DifferentiatorOutMin=[]  DifferentiatorOutMax=[]  FilterDiffOutCoefMin=[]  FilterDiffOutCoefMax=[]  ReciprocalOutMin=[]  ReciprocalOutMax=[]  SumDenOutMin=[]  SumDenOutMax=[]  SumNumOutMin=[]  SumNumOutMax=[]  DivideOutMin=[]  DivideOutMax=[]  UdiffTsProdOutMin=[]  UdiffTsProdOutMax=[]  NTsProdOutMin=[]  NTsProdOutMax=[]  UintegralTsProdOutMin=[]  UintegralTsProdOutMax=[]  UngainTsProdOutMin=[]  UngainTsProdOutMax=[]  ClampingZeroOutDataTypeStr=Inherit: Inherit via back propagation  ClampingZeroOutMin=[]  ClampingZeroOutMax=[]  FilterDenConstantOutDataTypeStr=Inherit: Inherit via back propagation  FilterDenConstantOutMin=[]  FilterDenConstantOutMax=[]  PCopyOutDataTypeStr=Inherit: Inherit via back propagation  PCopyOutMin=[]  PCopyOutMax=[]  NCopyOutDataTypeStr=Inherit: Inherit via back propagation  NCopyOutMin=[]  NCopyOutMax=[]  IntegratorContinuousStateAttributes=''  IntegratorStateMustResolveToSignalObject=off  IntegratorRTWStateStorageClass=Auto  FilterContinuousStateAttributes=''  FilterStateMustResolveToSignalObject=off  FilterRTWStateStorageClass=Auto  ParallelPVariant=Passthrough  IdealPVariant=InternalParameters  IVariant=InternalParameters  DVariant=InternalParameters  IntegratorVariant=Discrete  SatVariant=Enabled  AWVariant=DiscClampingIdeal  PCopyVariant=InternalParamsIdeal  TRVariant=Disabled  FdbkBlocksVariant=Forward  IdealPFdbkVariant=Disabled  SatFdbkVariant=Disabled  DerivativeFilterVariant=ForwardEulerFilter  NVariant=InternalParameters  NCopyVariant=Disabled  FilterICVariant=InternalICsFilter  IntegratorICVariant=InternalICs  ExternalResetVariant=Disabled  TRSumVariant=Passthrough  SumFdbkVariant=Disabled  SumVariant=Sum_PID  TsampFilterVariant=InternalTs  TsampNgainVariant=Passthrough  TsampIntegralVariant=Disabled_SignalSpec  ExternalSaturationOutDataTypeStr=Inherit: Same as second input
  Sum : Sum  Inputs=-+
  wrapTo180 : MATLAB Function  TreatAsAtomicUnit=on
      settings: MinAlgLoopOccurrences=on
  wrist_decoupler : Subsystem  TreatAsAtomicUnit=on  SystemSampleTime=0.001
      settings: MinAlgLoopOccurrences=on
  Tau* : Outport
  ypr_meas : Outport  Port=2
  Singularity : Outport  Port=3
  InRange : Outport  Port=4
  Cycles : Outport  Port=5
  wires:
  Sum/1 -> wrapTo180/1(u)
  wrapTo180/1(y) -> PID Controller/1
  PID Controller/1 -> Tau*/1
  theta_meas/1 -> wrist_decoupler/1(theta_meas), Sum/1
  ypr_star/1 -> wrist_decoupler/2(ypr_star)
  wrist_decoupler/1(theta_star) -> Sum/2
  wrist_decoupler/2(out_of_range) -> InRange/1
  wrist_decoupler/3(ypr_meas) -> ypr_meas/1
  wrist_decoupler/4(singularity) -> Singularity/1
  wrist_decoupler/5(cycles) -> Cycles/1

== system spherical_wrist/Simple Motor 1 ==
  Tau* : Inport
  Ideal Torque Source : fl_lib/Mechanical/Mechanical Sources/Ideal Torque Source
  Inertia2 : fl_lib/Mechanical/Rotational Elements/Inertia  inertia=Jm g*cm^2  num_ports=foundation.enum.numPorts2.one  w_specify=off  w_priority=High  w=0 rad/s  w_nominal_specify=off  w_nominal_unit=rad/s  w_nominal_value=1  t_specify=off  t_priority=None  t=0 N*m  t_nominal_specify=off  t_nominal_unit=N*m  t_nominal_value=1
  Rotational Damper : sdl_lib/Couplings & Drives/Springs & Dampers/Rotational Damper  D=Dm m*mN/rpm  enable_faults=0  b_fault=100 N*m/(rad/s)  temporal_fault=0  fault_time=5 s  shock_fault=0  acceleration_limit=100 rad/s^2  shock_limit=1  report_fault=(1)-1  thermal_port=simscape.enum.thermaleffects.omit  thermal_mass=50 kJ/K  temperature_specify=off  temperature_priority=High  temperature=300 K  temperature_nominal_specify=off  temperature_nominal_unit=K  temperature_nominal_value=1
  Simulink-PS Converter : nesl_utility/Simulink-PS Converter  PhysicalDomain=network_engine_domain  SubClassName=ps_input  LeftPortType=input  RightPortType=output  PseudoPeriodic=off  Frequencies=[]  NoiseDistribution=none  NoiseParameters=[]  Unit=N*m  AffineConversion=off  FilteringAndDerivatives=provide  SimscapeFilterOrder=2  InputFilterTimeConstant=0.001  UdotUserProvided=0
  R : PMIOPort  Side=Right
  C : PMIOPort  Port=2  Side=Right
  wires:
  Tau*/1 -> Simulink-PS Converter/1
  connections:
  Simulink-PS Converter/RConn1 -- Ideal Torque Source/RConn1
  Inertia2/LConn1 -- R/RConn1 -- Ideal Torque Source/LConn1 -- Rotational Damper/RConn1
  Ideal Torque Source/RConn2 -- C/RConn1 -- Rotational Damper/LConn1

== system spherical_wrist/Simple Motor 2 ==
  Tau* : Inport
  Ideal Torque Source : fl_lib/Mechanical/Mechanical Sources/Ideal Torque Source
  Inertia2 : fl_lib/Mechanical/Rotational Elements/Inertia  inertia=Jm g*cm^2  num_ports=foundation.enum.numPorts2.one  w_specify=off  w_priority=High  w=0 rad/s  w_nominal_specify=off  w_nominal_unit=rad/s  w_nominal_value=1  t_specify=off  t_priority=None  t=0 N*m  t_nominal_specify=off  t_nominal_unit=N*m  t_nominal_value=1
  Rotational Damper : sdl_lib/Couplings & Drives/Springs & Dampers/Rotational Damper  D=Dm m*mN/rpm  enable_faults=0  b_fault=100 N*m/(rad/s)  temporal_fault=0  fault_time=5 s  shock_fault=0  acceleration_limit=100 rad/s^2  shock_limit=1  report_fault=(1)-1  thermal_port=simscape.enum.thermaleffects.omit  thermal_mass=50 kJ/K  temperature_specify=off  temperature_priority=High  temperature=300 K  temperature_nominal_specify=off  temperature_nominal_unit=K  temperature_nominal_value=1
  Simulink-PS Converter : nesl_utility/Simulink-PS Converter  PhysicalDomain=network_engine_domain  SubClassName=ps_input  LeftPortType=input  RightPortType=output  PseudoPeriodic=off  Frequencies=[]  NoiseDistribution=none  NoiseParameters=[]  Unit=N*m  AffineConversion=off  FilteringAndDerivatives=provide  SimscapeFilterOrder=2  InputFilterTimeConstant=0.001  UdotUserProvided=0
  R : PMIOPort  Side=Right
  C : PMIOPort  Port=2  Side=Right
  wires:
  Tau*/1 -> Simulink-PS Converter/1
  connections:
  Simulink-PS Converter/RConn1 -- Ideal Torque Source/RConn1
  Ideal Torque Source/LConn1 -- Inertia2/LConn1 -- Rotational Damper/RConn1 -- R/RConn1
  Rotational Damper/LConn1 -- Ideal Torque Source/RConn2 -- C/RConn1

== system spherical_wrist/Simple Motor 3 ==
  Tau* : Inport
  Ideal Torque Source : fl_lib/Mechanical/Mechanical Sources/Ideal Torque Source
  Inertia2 : fl_lib/Mechanical/Rotational Elements/Inertia  inertia=Jm g*cm^2  num_ports=foundation.enum.numPorts2.one  w_specify=off  w_priority=High  w=0 rad/s  w_nominal_specify=off  w_nominal_unit=rad/s  w_nominal_value=1  t_specify=off  t_priority=None  t=0 N*m  t_nominal_specify=off  t_nominal_unit=N*m  t_nominal_value=1
  Rotational Damper : sdl_lib/Couplings & Drives/Springs & Dampers/Rotational Damper  D=Dm m*mN/rpm  enable_faults=0  b_fault=100 N*m/(rad/s)  temporal_fault=0  fault_time=5 s  shock_fault=0  acceleration_limit=100 rad/s^2  shock_limit=1  report_fault=(1)-1  thermal_port=simscape.enum.thermaleffects.omit  thermal_mass=50 kJ/K  temperature_specify=off  temperature_priority=High  temperature=300 K  temperature_nominal_specify=off  temperature_nominal_unit=K  temperature_nominal_value=1
  Simulink-PS Converter : nesl_utility/Simulink-PS Converter  PhysicalDomain=network_engine_domain  SubClassName=ps_input  LeftPortType=input  RightPortType=output  PseudoPeriodic=off  Frequencies=[]  NoiseDistribution=none  NoiseParameters=[]  Unit=N*m  AffineConversion=off  FilteringAndDerivatives=provide  SimscapeFilterOrder=2  InputFilterTimeConstant=0.001  UdotUserProvided=0
  R : PMIOPort  Side=Right
  C : PMIOPort  Port=2  Side=Right
  wires:
  Tau*/1 -> Simulink-PS Converter/1
  connections:
  Simulink-PS Converter/RConn1 -- Ideal Torque Source/RConn1
  Ideal Torque Source/LConn1 -- Inertia2/LConn1 -- Rotational Damper/RConn1 -- R/RConn1
  Rotational Damper/LConn1 -- Ideal Torque Source/RConn2 -- C/RConn1
